simulink model "T10_Sim_BPSK_1"  (R2015a)
settings: Solver=ode45  StartTime=0.0  StopTime=10.0  RelTol=1e-3
libraries: commdigbbndpm3 x2, commrandsrc2 x1
settings Model: Creator=User  LastModifiedBy=User

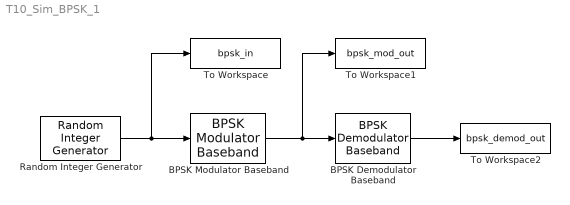
== system T10_Sim_BPSK_1 ==
  BPSK Demodulator Baseband : commdigbbndpm3/BPSK Demodulator Baseband  Ph=0  DecType=Hard decision  VarSource=Dialog  Variance=1  outDtype=Inherit via internal rule  derotateFactorWordLen=16
  BPSK Modulator Baseband : commdigbbndpm3/BPSK Modulator Baseband  Ph=0  outDtype=double  outWordLen=16  outUDDataType=sfix(16)  outFracLenMode=Best precision  outFracLen=15
  Random Integer Generator : commrandsrc2/Random Integer Generator  mul=2  seed=37  Ts=1  frameBased=off  sampPerFrame=1000  orient=off  outDataType=boolean
  To Workspace : ToWorkspace  VariableName=bpsk_in  SaveFormat=Timeseries  SampleTime=-1
  To Workspace1 : ToWorkspace  VariableName=bpsk_mod_out  SaveFormat=Timeseries  SampleTime=-1
  To Workspace2 : ToWorkspace  VariableName=bpsk_demod_out  SaveFormat=Timeseries  SampleTime=-1
  wires:
  Random Integer Generator/1 -> To Workspace/1, BPSK Modulator Baseband/1
  BPSK Modulator Baseband/1 -> To Workspace1/1, BPSK Demodulator Baseband/1
  BPSK Demodulator Baseband/1 -> To Workspace2/1
